simulink subsystem "Subsys_GFormConv_OuterCtrl_Dual_Port"  (R2022b)
settings: Solver=VariableStepAuto  StartTime=0.0  StopTime=1  RelTol=1e-3
model mask{f_n=50, K_p=0.01, K_d=1e-4, s_droop_QV=0.1, T_Q=0.2, T_s_ctrl=1e-3, T_s_PWM_meas=1e-4}
  mask prompts: f_n "Nominal frequency [Hz]"; K_p "Proportional gain [pu]"; K_d "Derivative gain [pu]"; s_droop_QV "Droop constant kQ (dV[pu]/dQ[pu])"; T_Q "PT1 time constant (for QV control) [s]"; T_s_ctrl "Controller sample time [s]"; T_s_PWM_meas "PWM and measurements sample time [s]"
undefined symbols (not defined in the file): alpha_LPF_Q
libraries: simulink x1, slpidlib x1
settings Model: DefaultTestHarness=Subsys_GFormConv_OuterCtrl_Dual_Port_Harness  Creator=j.jansen  LastModifiedBy=pc236admin

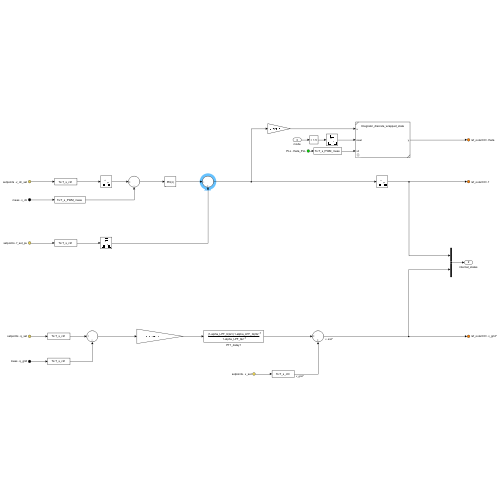
[thumbnail: Simulink's stored preview of the top-level diagram]
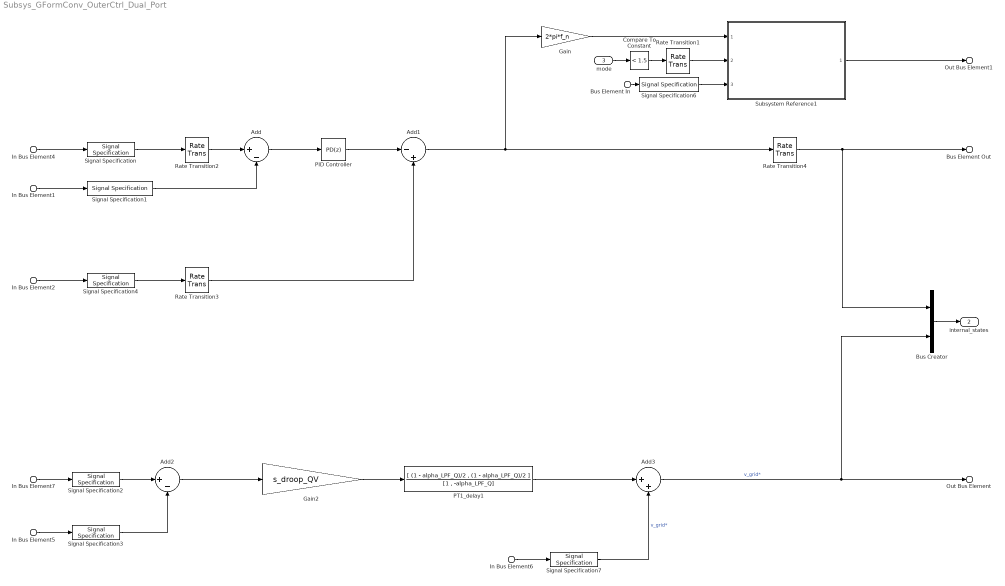
== system Subsys_GFormConv_OuterCtrl_Dual_Port ==
  In Bus Element2 : Inport  PortName=setpoints  Element=f_set_pu
  In Bus Element4 : Inport  PortName=setpoints  Element=v_dc_set
  In Bus Element6 : Inport  PortName=setpoints  Element=v_set
  In Bus Element7 : Inport  PortName=setpoints  Element=q_set
  In Bus Element1 : Inport  Port=2  PortName=meas  Element=v_dc
  In Bus Element5 : Inport  Port=2  PortName=meas  Element=q_grid
  mode : Inport  Port=3
  Bus Element In : Inport  Port=4  PortName=PLL  Element=theta_PLL
  Add : Sum  Inputs=|+-
  Add1 : Sum  Inputs=|-+
  Add2 : Sum  Inputs=|+-
  Add3 : Sum  Inputs=|++
  Bus Creator : BusCreator  Inputs=2
  Compare To Constant : simulink/Logic and Bit Operations/Compare To Constant  relop=<  const=1.5  OutDataTypeStr=boolean
  Gain : Gain  Gain=2*pi*f_n
  Gain2 : Gain  Gain=s_droop_QV
  PID Controller : slpidlib/PID Controller  Controller=PD  Form=Parallel  TimeDomain=Discrete-time  UseExternalTs=off  SampleTime=T_s_PWM_meas  IntegratorMethod=Forward Euler  FilterMethod=Forward Euler  ControllerParametersSource=internal  P=K_p  I=0.5  UseKiTs=off  D=K_d  N=100  UseFilter=on  TunerSelectOption=Transfer Function Based (PID Tuner App)  InitialConditionSource=internal  InitialConditionForIntegrator=0  InitialConditionForFilter=0  DifferentiatorICPrevScaledInput=0  ExternalReset=none  TrackingMode=off  Kt=1  LimitOutput=off  SatLimitsSource=internal  UpperSaturationLimit=2*pi  LowerSaturationLimit=0  LinearizeAsGain=on  AntiWindupMode=clamping  Kb=1  LimitIntegrator=off  UpperIntegratorSaturationLimit=0  LowerIntegratorSaturationLimit=2*pi  POutMin=[]  POutMax=[]  IOutMin=[]  IOutMax=[]  DOutMin=[]  DOutMax=[]  NOutMin=[]  NOutMax=[]  SumOutMin=[]  SumOutMax=[]  SaturationOutMin=[]  SaturationOutMax=[]  PParamMin=[]  PParamMax=[]  IParamMin=[]  IParamMax=[]  DParamMin=[]  DParamMax=[]  NParamMin=[]  NParamMax=[]  KbParamMin=[]  KbParamMax=[]  KtParamMin=[]  KtParamMax=[]  KbOutMin=[]  KbOutMax=[]  KtOutMin=[]  KtOutMax=[]  IntegratorOutMin=[]  IntegratorOutMax=[]  FilterOutMin=[]  FilterOutMax=[]  SumI1OutMin=[]  SumI1OutMax=[]  SumI2OutMin=[]  SumI2OutMax=[]  SumI3OutMin=[]  SumI3OutMax=[]  SumI4OutMin=[]  SumI4OutMax=[]  SumDOutMin=[]  SumDOutMax=[]  DifferentiatorOutMin=[]  DifferentiatorOutMax=[]  FilterDiffOutCoefMin=[]  FilterDiffOutCoefMax=[]  ReciprocalOutMin=[]  ReciprocalOutMax=[]  SumDenOutMin=[]  SumDenOutMax=[]  SumNumOutMin=[]  SumNumOutMax=[]  DivideOutMin=[]  DivideOutMax=[]  UdiffTsProdOutMin=[]  UdiffTsProdOutMax=[]  NTsProdOutMin=[]  NTsProdOutMax=[]  UintegralTsProdOutMin=[]  UintegralTsProdOutMax=[]  UngainTsProdOutMin=[]  UngainTsProdOutMax=[]  ClampingZeroOutDataTypeStr=Inherit: Inherit via back propagation  ClampingZeroOutMin=[]  ClampingZeroOutMax=[]  FilterDenConstantOutDataTypeStr=Inherit: Inherit via back propagation  FilterDenConstantOutMin=[]  FilterDenConstantOutMax=[]  PCopyOutDataTypeStr=Inherit: Inherit via back propagation  PCopyOutMin=[]  PCopyOutMax=[]  NCopyOutDataTypeStr=Inherit: Inherit via back propagation  NCopyOutMin=[]  NCopyOutMax=[]  IntegratorContinuousStateAttributes=''  IntegratorStateMustResolveToSignalObject=off  IntegratorRTWStateStorageClass=Auto  FilterContinuousStateAttributes=''  FilterStateMustResolveToSignalObject=off  FilterRTWStateStorageClass=Auto  ParallelPVariant=InternalParameters  IdealPVariant=Disabled  IVariant=Disabled  DVariant=InternalParameters  IntegratorVariant=Disabled  SatVariant=Disabled  AWVariant=Disabled  PCopyVariant=Disabled  TRVariant=Disabled  FdbkBlocksVariant=Forward  IdealPFdbkVariant=Disabled  SatFdbkVariant=Disabled  DerivativeFilterVariant=ForwardEulerFilter  NVariant=InternalParameters  NCopyVariant=Disabled  FilterICVariant=InternalICsFilter  IntegratorICVariant=Disabled  ExternalResetVariant=Disabled  TRSumVariant=Passthrough  SumFdbkVariant=Disabled  SumVariant=Sum_PD  TsampFilterVariant=InternalTs  TsampNgainVariant=Passthrough  TsampIntegralVariant=Disabled_SignalSpec  ExternalSaturationOutDataTypeStr=Inherit: Same as second input
  PT1_delay1 : DiscreteFilter  Numerator=[ (1 - alpha_LPF_Q)/2 , (1 - alpha_LPF_Q)/2 ]  Denominator=[1 , -alpha_LPF_Q]  SampleTime=T_s_ctrl
  Rate Transition1 : RateTransition  Deterministic=off  OutPortSampleTime=T_s_PWM_meas
  Rate Transition2 : RateTransition  Deterministic=off  OutPortSampleTime=T_s_PWM_meas
  Rate Transition3 : RateTransition  Deterministic=off  OutPortSampleTime=T_s_PWM_meas
  Rate Transition4 : RateTransition  Deterministic=off  OutPortSampleTime=T_s_ctrl
  Signal Specification{,2..4,7} (5 alike) : SignalSpecification  SampleTime=T_s_ctrl
  Signal Specification1 : SignalSpecification  SampleTime=T_s_PWM_meas
  Signal Specification6 : SignalSpecification  SampleTime=T_s_PWM_meas
  Subsystem Reference1 : Subsystem  ReferencedSubsystem=Integrator_discrete_wrapped_state  WrappedStateUpperValue=2*pi  WrappedStateLowerValue=0  x_0=0  T_s=T_s_PWM_meas
  Bus Element Out : Outport  PortName=ref_outerCtrl  Element=f
  Out Bus Element1 : Outport  PortName=ref_outerCtrl  Element=theta
  Out Bus Element : Outport  PortName=ref_outerCtrl  Element=v_grid*
  internal_states : Outport  Port=2
  wires:
  Bus Creator/1 -> internal_states/1
  Add/1 -> PID Controller/1
  Add1/1 -> Gain/1, Rate Transition4/1
  mode/1 -> Compare To Constant/1
  Signal Specification6/1 -> Subsystem Reference1/3
  Gain/1 -> Subsystem Reference1/1
  Bus Element In/1 -> Signal Specification6/1
  Rate Transition1/1 -> Subsystem Reference1/2
  Signal Specification4/1 -> Rate Transition3/1
  Compare To Constant/1 -> Rate Transition1/1
  In Bus Element2/1 -> Signal Specification4/1
  PID Controller/1 -> Add1/1
  Signal Specification1/1 -> Add/2
  In Bus Element1/1 -> Signal Specification1/1
  In Bus Element4/1 -> Signal Specification/1
  Signal Specification/1 -> Rate Transition2/1
  In Bus Element6/1 -> Signal Specification7/1
  Signal Specification2/1 -> Add2/1
  Add3/1 -> Bus Creator/2, Out Bus Element/1  "v_grid*"
  Signal Specification7/1 -> Add3/2  "v_grid*"
  In Bus Element7/1 -> Signal Specification2/1
  In Bus Element5/1 -> Signal Specification3/1
  Signal Specification3/1 -> Add2/2
  PT1_delay1/1 -> Add3/1
  Gain2/1 -> PT1_delay1/1
  Add2/1 -> Gain2/1
  Subsystem Reference1/1 -> Out Bus Element1/1
  Rate Transition2/1 -> Add/1
  Rate Transition3/1 -> Add1/2
  Rate Transition4/1 -> Bus Creator/1, Bus Element Out/1
